simulink model "diode_rectifier"  (R2021a)
settings: Solver=VariableStepAuto  StartTime=0.0  StopTime=0.08  RelTol=1e-3
libraries: spsDiodeLib x9, spsSeriesRLCBranchLib x8, spsACVoltageSourceLib x6, spsCurrentMeasurementLib x2, spsMeanLib x2, spsVoltageMeasurementLib x2, spspowerguiLib x1
settings Model: Creator=lenovo  LastModifiedBy=lenovo

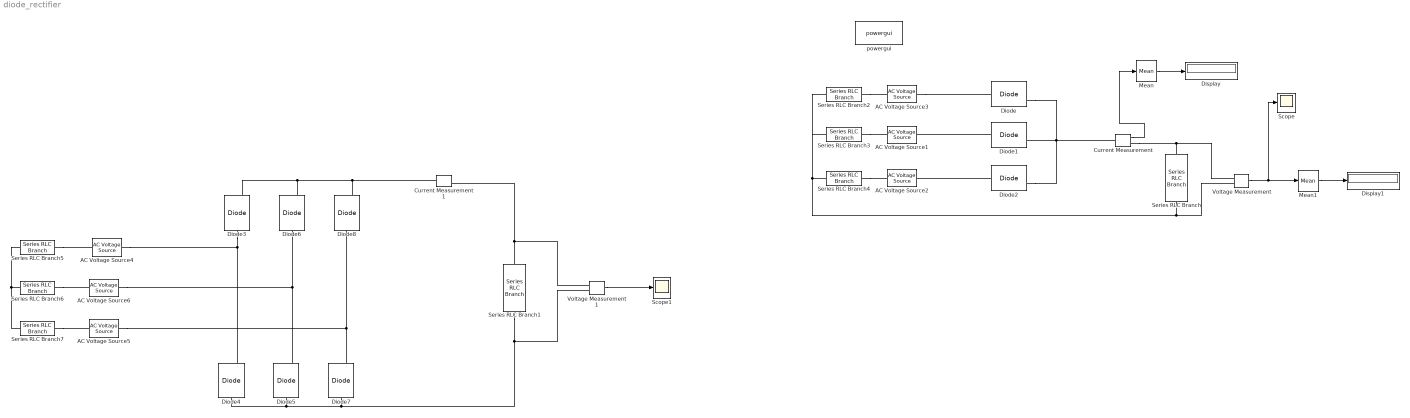
== system diode_rectifier ==
  AC Voltage Source1 : spsACVoltageSourceLib/AC Voltage Source  Amplitude=sqrt(2)*135  Phase=-120  Frequency=50  SampleTime=0  Measurements=None  BusType=swing  Pref=10e3  Qref=0  Qmin=-inf  Qmax=+inf
  AC Voltage Source2 : spsACVoltageSourceLib/AC Voltage Source  Amplitude=sqrt(2)*135  Phase=-240  Frequency=50  SampleTime=0  Measurements=None  BusType=swing  Pref=10e3  Qref=0  Qmin=-inf  Qmax=+inf
  AC Voltage Source3 : spsACVoltageSourceLib/AC Voltage Source  Amplitude=sqrt(2)*135  Phase=0  Frequency=50  SampleTime=0  Measurements=None  BusType=swing  Pref=10e3  Qref=0  Qmin=-inf  Qmax=+inf
  AC Voltage Source4 : spsACVoltageSourceLib/AC Voltage Source  Amplitude=sqrt(2)*135  Phase=0  Frequency=50  SampleTime=0  Measurements=None  BusType=swing  Pref=10e3  Qref=0  Qmin=-inf  Qmax=+inf
  AC Voltage Source5 : spsACVoltageSourceLib/AC Voltage Source  Amplitude=sqrt(2)*135  Phase=-240  Frequency=50  SampleTime=0  Measurements=None  BusType=swing  Pref=10e3  Qref=0  Qmin=-inf  Qmax=+inf
  AC Voltage Source6 : spsACVoltageSourceLib/AC Voltage Source  Amplitude=sqrt(2)*135  Phase=-120  Frequency=50  SampleTime=0  Measurements=None  BusType=swing  Pref=10e3  Qref=0  Qmin=-inf  Qmax=+inf
  Current Measurement : spsCurrentMeasurementLib/Current Measurement  PhasorSimulation=off  OutputType=Complex  PSBequivalent=0
  Current Measurement1 : spsCurrentMeasurementLib/Current Measurement  PhasorSimulation=off  OutputType=Complex  PSBequivalent=0
  Diode{,1..8} (9 alike) : spsDiodeLib/Diode  Ron=0.001  Lon=0  Vf=0.8  IC=0  UseSnubber=0  Rs=500  Cs=250e-9  Measurements=on
  Display : Display
  Display1 : Display
  Mean : spsMeanLib/Mean  Freq=60  Vinit=0  Ts=0
  Mean1 : spsMeanLib/Mean  Freq=60  Vinit=0  Ts=0
  Scope : Scope
  Scope1 : Scope
  Series RLC Branch : spsSeriesRLCBranchLib/Series RLC Branch  LConnTagsString=__new0  RConnTagsString=__new0  BranchType=RL  Resistance=54  Inductance=0.189  SetiL0=off  InitialCurrent=0  Capacitance=1e-6  Setx0=off  InitialVoltage=0  Measurements=None
  Series RLC Branch1 : spsSeriesRLCBranchLib/Series RLC Branch  LConnTagsString=__new0  RConnTagsString=__new0  BranchType=RL  Resistance=1  Inductance=1e-3  SetiL0=off  InitialCurrent=0  Capacitance=1e-6  Setx0=off  InitialVoltage=0  Measurements=None
  Series RLC Branch2 : spsSeriesRLCBranchLib/Series RLC Branch  LConnTagsString=__new0  RConnTagsString=__new0  BranchType=L  Resistance=1  Inductance=1e-4  SetiL0=off  InitialCurrent=0  Capacitance=1e-6  Setx0=off  InitialVoltage=0  Measurements=None
  Series RLC Branch3 : spsSeriesRLCBranchLib/Series RLC Branch  LConnTagsString=__new0  RConnTagsString=__new0  BranchType=L  Resistance=1  Inductance=1e-4  SetiL0=off  InitialCurrent=0  Capacitance=1e-6  Setx0=off  InitialVoltage=0  Measurements=None
  Series RLC Branch4 : spsSeriesRLCBranchLib/Series RLC Branch  LConnTagsString=__new0  RConnTagsString=__new0  BranchType=L  Resistance=1  Inductance=1e-4  SetiL0=off  InitialCurrent=0  Capacitance=1e-6  Setx0=off  InitialVoltage=0  Measurements=None
  Series RLC Branch5 : spsSeriesRLCBranchLib/Series RLC Branch  LConnTagsString=__new0  RConnTagsString=__new0  BranchType=L  Resistance=1  Inductance=1e-6  SetiL0=off  InitialCurrent=0  Capacitance=1e-6  Setx0=off  InitialVoltage=0  Measurements=None
  Series RLC Branch6 : spsSeriesRLCBranchLib/Series RLC Branch  LConnTagsString=__new0  RConnTagsString=__new0  BranchType=L  Resistance=1  Inductance=1e-6  SetiL0=off  InitialCurrent=0  Capacitance=1e-6  Setx0=off  InitialVoltage=0  Measurements=None
  Series RLC Branch7 : spsSeriesRLCBranchLib/Series RLC Branch  LConnTagsString=__new0  RConnTagsString=__new0  BranchType=L  Resistance=1  Inductance=1e-6  SetiL0=off  InitialCurrent=0  Capacitance=1e-6  Setx0=off  InitialVoltage=0  Measurements=None
  Voltage Measurement : spsVoltageMeasurementLib/Voltage Measurement  PhasorSimulation=off  OutputType=Complex  PSBequivalent=0
  Voltage Measurement1 : spsVoltageMeasurementLib/Voltage Measurement  PhasorSimulation=off  OutputType=Complex  PSBequivalent=0
  powergui : spspowerguiLib/powergui  Priority=1  SimulationMode=Continuous  SampleTime=50e-6  frequency=60  Iterations=50  frequencyindice=50  Pbase=100e6  ErrMax=1e-4  UnitsV=kV  UnitsW=MW  buscounter=0  FunctionMessages=off  echomessages=off  EnableUseOfTLC=off  CurrentSourceSwitches=off  DisableSnubberDevices=off  DisableRonSwitches=off  DisableVfSwitches=off  DisplayEquations=off  AutomaticDiscreteSolvers=off  SolverType=Tustin/Backward Euler (TBE)  Interpol=off  ExternalGateDelay=off  methode=off  Ts=100  x0status=blocks  SPID=on  SwTol=0  HookPort=off  NonlinearTolerance=1e-4  nMaxIteration=100  ContinueOnMaxIteration=off  RestoreLinks=warning  ResistiveCurrentMeasurement=off  Frange=[0:2:500]  Ylog=off  Xlog=on  ShowGrid=off  save=off  variable=ZData  structure=0  ZoomFFT=off  StartTime=0.0  cycles=1  DisplayStyle=1  fundamental=60  FreqAxis=off  MaxFrequency=1000  frequencyindicesteady=1  RmsSteady=1  display=off
  wires:
  Voltage Measurement/1 -> Scope/1, Mean1/1
  Mean/1 -> Display/1
  Mean1/1 -> Display1/1
  Current Measurement/1 -> Mean/1
  Voltage Measurement1/1 -> Scope1/1
  connections:
  AC Voltage Source3/RConn1 -- Diode/LConn1
  Diode2/LConn1 -- AC Voltage Source2/RConn1
  Diode1/LConn1 -- AC Voltage Source1/RConn1
  Series RLC Branch/LConn1 -- Current Measurement/RConn1 -- Voltage Measurement/LConn1
  Diode5/RConn1 -- AC Voltage Source6/RConn1 -- Diode6/LConn1
  Diode3/LConn1 -- Diode4/RConn1 -- AC Voltage Source4/RConn1
  Diode7/RConn1 -- AC Voltage Source5/RConn1 -- Diode8/LConn1
  Current Measurement1/LConn1 -- Diode8/RConn1 -- Diode6/RConn1 -- Diode3/RConn1
  Series RLC Branch1/LConn1 -- Voltage Measurement1/LConn1 -- Current Measurement1/RConn1
  Series RLC Branch1/RConn1 -- Voltage Measurement1/LConn2 -- Diode7/LConn1 -- Diode5/LConn1 -- Diode4/LConn1
  Voltage Measurement/LConn2 -- Series RLC Branch3/LConn1 -- Series RLC Branch2/LConn1 -- Series RLC Branch4/LConn1 -- Series RLC Branch/RConn1
  Diode2/RConn1 -- Diode/RConn1 -- Current Measurement/LConn1 -- Diode1/RConn1
  Series RLC Branch2/RConn1 -- AC Voltage Source3/LConn1
  Series RLC Branch4/RConn1 -- AC Voltage Source2/LConn1
  Series RLC Branch3/RConn1 -- AC Voltage Source1/LConn1
  Series RLC Branch5/RConn1 -- AC Voltage Source4/LConn1
  Series RLC Branch7/RConn1 -- AC Voltage Source5/LConn1
  Series RLC Branch6/RConn1 -- AC Voltage Source6/LConn1
  Series RLC Branch5/LConn1 -- Series RLC Branch7/LConn1 -- Series RLC Branch6/LConn1
